simulink model "Simulink"  (R2024b)
settings: Solver=ode4  StartTime=0.0  StopTime=20  FixedStep=0.001  RelTol=1e-6
settings Model: LastModifiedBy=Manu

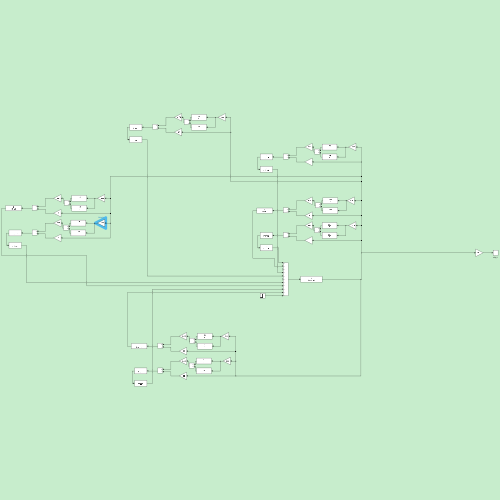
[thumbnail: Simulink's stored preview of the top-level diagram]
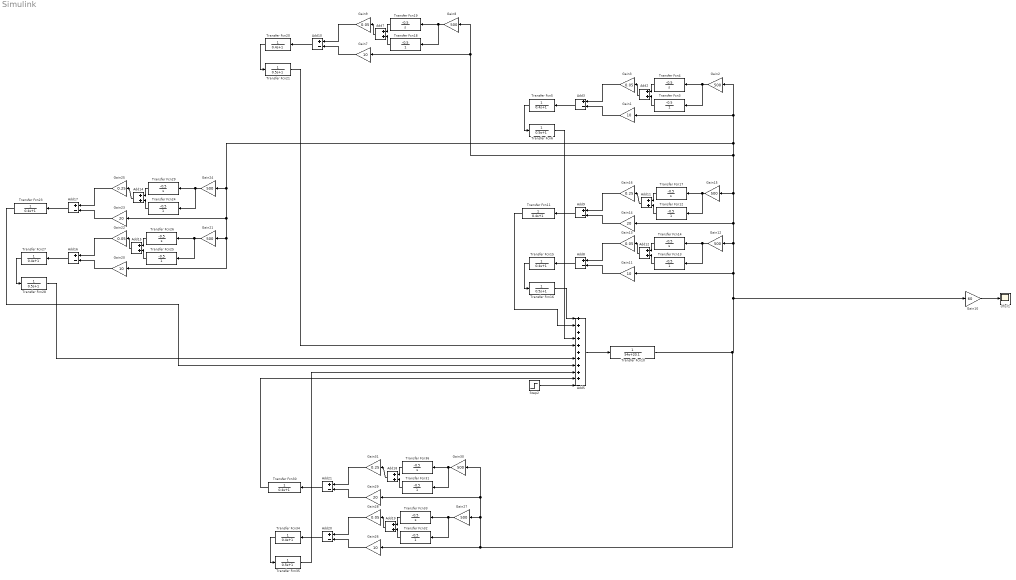
== system Simulink ==
  Add{3,8..10,16..17,20..21} (8 alike) : Sum  Inputs=+-
  Add{2,7,11..12,14..15,18..19} (8 alike) : Sum
  Add5 : Sum  Inputs=++++++++++-
  Gain{1,7,11,20,26} (5 alike) : Gain  Gain=10
  Gain10 : Gain  Gain=60
  Gain{2,8,12,15,21,24,27,30} (8 alike) : Gain  Gain=500
  Gain{3,9,13,22,28} (5 alike) : Gain  Gain=0.05
  Gain14 : Gain  Gain=20
  Gain16 : Gain  Gain=0.25
  Gain23 : Gain  Gain=20
  Gain25 : Gain  Gain=0.25
  Gain29 : Gain  Gain=20
  Gain31 : Gain  Gain=0.25
  Step2 : Step  Time=0  After=0.1  SampleTime=0
  Transfer Fcn10 : TransferFcn  Denominator=[54 20.1]
  Transfer Fcn{5,11,15,20,23,27,30,34} (8 alike) : TransferFcn  Denominator=[0.4,1]
  Transfer Fcn{3,12..13,18,24..25,31..32} (8 alike) : TransferFcn  Numerator=[0,-0.5]  Denominator=[0,1]
  Transfer Fcn{4,14,17,19,26,29,33,36} (8 alike) : TransferFcn  Numerator=[0,-0.5]  Denominator=[1,0]
  Transfer Fcn{6,16,21,28,35} (5 alike) : TransferFcn  Denominator=[0.5,1]
  df(s)1 : Scope
  wires:
  Gain15/1 -> Transfer Fcn12/1, Transfer Fcn17/1
  Transfer Fcn14/1 -> Add12/1
  Gain12/1 -> Transfer Fcn13/1, Transfer Fcn14/1
  Add8/1 -> Transfer Fcn15/1
  Add12/1 -> Gain13/1
  Transfer Fcn13/1 -> Add12/2
  Transfer Fcn15/1 -> Transfer Fcn16/1
  Transfer Fcn16/1 -> Add5/1
  Add11/1 -> Gain16/1
  Gain16/1 -> Add9/1
  Gain13/1 -> Add8/1
  Transfer Fcn11/1 -> Add5/2
  Gain14/1 -> Add9/2
  Add5/1 -> Transfer Fcn10/1
  Transfer Fcn17/1 -> Add11/1
  Gain10/1 -> df(s)1/1
  Transfer Fcn12/1 -> Add11/2
  Gain11/1 -> Add8/2
  Add9/1 -> Transfer Fcn11/1
  Step2/1 -> Add5/11
  Add2/1 -> Gain3/1
  Add3/1 -> Transfer Fcn5/1
  Gain2/1 -> Transfer Fcn3/1, Transfer Fcn4/1
  Transfer Fcn6/1 -> Add5/4
  Transfer Fcn4/1 -> Add2/1
  Transfer Fcn3/1 -> Add2/2
  Transfer Fcn5/1 -> Transfer Fcn6/1
  Gain3/1 -> Add3/1
  Gain1/1 -> Add3/2
  Transfer Fcn21/1 -> Add5/5
  Add10/1 -> Transfer Fcn20/1
  Gain8/1 -> Transfer Fcn18/1, Transfer Fcn19/1
  Transfer Fcn19/1 -> Add7/1
  Gain7/1 -> Add10/2
  Gain9/1 -> Add10/1
  Add7/1 -> Gain9/1
  Transfer Fcn20/1 -> Transfer Fcn21/1
  Transfer Fcn18/1 -> Add7/2
  Transfer Fcn28/1 -> Add5/7
  Add16/1 -> Transfer Fcn27/1
  Gain21/1 -> Transfer Fcn25/1, Transfer Fcn26/1
  Transfer Fcn26/1 -> Add15/1
  Gain24/1 -> Transfer Fcn24/1, Transfer Fcn29/1
  Gain20/1 -> Add16/2
  Gain22/1 -> Add16/1
  Gain23/1 -> Add17/2
  Add15/1 -> Gain22/1
  Transfer Fcn27/1 -> Transfer Fcn28/1
  Transfer Fcn29/1 -> Add14/1
  Transfer Fcn24/1 -> Add14/2
  Transfer Fcn23/1 -> Add5/8
  Add17/1 -> Transfer Fcn23/1
  Add14/1 -> Gain25/1
  Gain25/1 -> Add17/1
  Transfer Fcn25/1 -> Add15/2
  Transfer Fcn35/1 -> Add5/9
  Add20/1 -> Transfer Fcn34/1
  Gain27/1 -> Transfer Fcn32/1, Transfer Fcn33/1
  Transfer Fcn33/1 -> Add19/1
  Gain30/1 -> Transfer Fcn31/1, Transfer Fcn36/1
  Gain26/1 -> Add20/2
  Gain28/1 -> Add20/1
  Gain29/1 -> Add21/2
  Add19/1 -> Gain28/1
  Transfer Fcn34/1 -> Transfer Fcn35/1
  Transfer Fcn36/1 -> Add18/1
  Transfer Fcn31/1 -> Add18/2
  Transfer Fcn30/1 -> Add5/10
  Add21/1 -> Transfer Fcn30/1
  Add18/1 -> Gain31/1
  Gain31/1 -> Add21/1
  Transfer Fcn10/1 -> Gain29/1, Gain30/1, Gain27/1, Gain26/1, Gain14/1, Gain8/1, Gain7/1, Gain20/1, Gain21/1, Gain23/1, Gain24/1, Gain2/1, Gain1/1, Gain15/1, Gain12/1, Gain11/1, Gain10/1
  Transfer Fcn32/1 -> Add19/2
